simulink library "Valve_Lib"  (R2025a)
settings: Solver=ode45  StartTime=0.0  StopTime=10.0  RelTol=1e-3  EnableMultiTasking=on
libraries: fl_lib x13, Custom_lib x2, SimscapeFluids_lib x1
Description:
  | Copyright 2015-2025 The MathWorks, Inc.
settings Model: Creator=smiller  LastModifiedBy=smiller
settings SolverCC: AlgebraicLoopSolver=TrustRegion
settings DataIOCC: LimitDataPoints=on  SaveFormat=Array  ReturnWorkspaceOutputs=off
settings OptimizationCC: ReuseModelBlockBuffer=off  ExpressionDepthLimit=2147483647.0  LifeSpan=inf
settings DebuggingCC: UnderspecifiedInitializationDetection=Classic  MergeDetectMultiDrivingBlocksExec=none  SolverPrmCheckMsg=warning  UnconnectedInputMsg=warning  UnconnectedOutputMsg=warning  UnconnectedLineMsg=warning  AllowSymbolicDim=off  StateNameClashWarn=warning  PregeneratedLibrarySubsystemCodeDiagnostic=none  SFUnexpectedBacktrackingDiag=warning  SFNoUnconditionalDefaultTransitionDiag=warning  SFExecutionAtInitializationDiag=none  ArithmeticOperatorsInVariantConditions=warning
settings HardwareCC: ProdBitPerPointer=32.0  ProdBitPerSizeT=32.0  ProdBitPerPtrDiffT=32.0  ProdLargestAtomicFloat=None  ProdIntDivRoundTo=Undefined  ProdEndianess=Unspecified  ProdWordSize=32.0  ProdHWDeviceType=32-bit Generic
settings ModelReferenceCC: EnableRefExpFcnMdlSchedulingChecks=on  PropagateSignalLabelsOutOfModel=off
settings SFSimCC: SimUseLocalCustomCode=off  CustomCodeUndefinedFunction=UseInterfaceOnly
settings RTWCC: RTWUseLocalCustomCode=off  GPUComputeCapability=3.5  DLArmComputeVersion=19.05
settings CodeAppCC: StateflowObjectComments=on
settings GRTTargetCC: TargetLangStandard=C89/C90 (ANSI)
settings ConfigComp: CovMetricSettings=dw  CovSaveCumulativeToWorkspaceVar=on  CovSaveSingleToWorkspaceVar=on  CovExternalEMLEnable=off  CovSFcnEnable=off

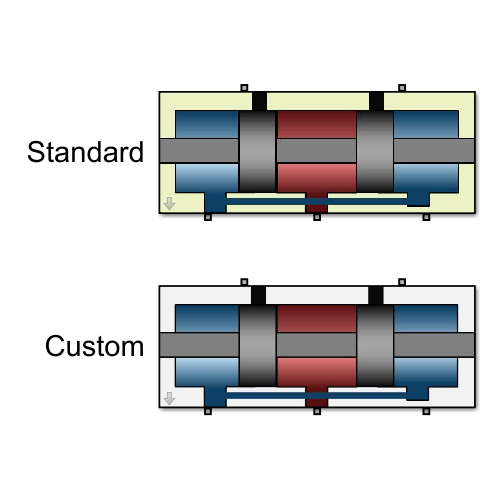
[thumbnail: Simulink's stored preview of the top-level diagram]
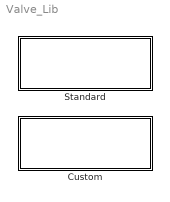
== system Valve_Lib ==
  Custom : Subsystem  VariantControl=Custom  mask(Single-Stage Servo Valve){K_V=0.5, x_max=0.5, A_max=9, x_lap=0.02, A_leak=0.25}
      mask prompts: K_V "Flow Coefficient:"; x_max "Spool travel limit (mm)"; A_max "Maximum orifice area (mm^2)"; x_lap "Spool travel with leakage (mm)"; A_leak "Leakage area at x=0 (mm^2)"
      mask help: Models a spool valve actuated directly by a torque motor using Simscape Foundation library components.
      mask Display: image('Four_Way_Valve_Custom_IMAGE.jpg')
  Standard : Subsystem  VariantControl=Standard  mask(Single-Stage Servo Valve){K_V=0.5, x_max=0.5, A_max=9, x_lap=0.02, A_leak=0.25}
      mask prompts: K_V "Flow Coefficient:"; x_max "Spool travel limit (mm)"; A_max "Maximum orifice area (mm^2)"; x_lap "Spool travel with leakage (mm)"; A_leak "Leakage area at x=0 (mm^2)"
      mask help: Models a spool valve actuated directly by a torque motor using Simscape add-on library components.
      mask Display: image(imread('Four_Way_Valve_Standard_IMAGE.jpg'))

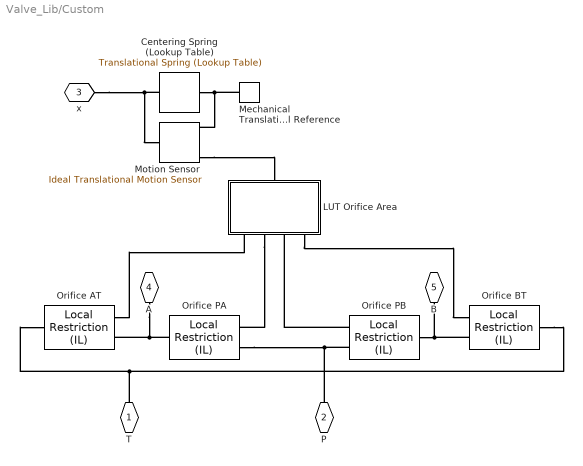
== system Valve_Lib/Custom ==
  Centering Spring (Lookup Table) : Custom_lib/Mechanical/Translational Spring (Lookup Table)  xd=[-1 -0.9 0,0.9 1]*x_max mm  kd=[100,10,10,10,100] N/m  f_specify=off  f_priority=High  f=0 N  f_nominal_specify=off  f_nominal_value=1  f_nominal_unit=N  x_specify=off  x_priority=High  x=0 m  x_nominal_specify=off  x_nominal_value=1  x_nominal_unit=m  v_specify=off  v_priority=High  v=0 m/s  v_nominal_specify=off  v_nominal_value=1  v_nominal_unit=m/s  k_specify=off  k_priority=High  k=0 N/m  k_nominal_specify=off  k_nominal_value=1  k_nominal_unit=N/m
      settings: InternalSimscapePortConfiguration="{\"Bottom\":[],\"Left\":[{\"id\":\"c\",\"label\":\"c\",\"type\":\"foundation.mechanical.translational.translational\"}],\"Right\":[{\"id\":\"r\",\"label\":\"r\",\"type\":\"foundation.mechanical.translational.translational\"}],\"Top\":[]}"
  LUT Orifice Area : Subsystem
  Mechanical Translational Reference : fl_lib/Mechanical/Translational Elements/Mechanical Translational Reference
  Motion Sensor : fl_lib/Mechanical/Mechanical Sensors/Ideal Translational Motion Sensor  reference=foundation.enum.MeasurementReference.difference  acceleration_port=false  velocity_port=true  position_port=true  offset=0 m
  Orifice AT : fl_lib/Isothermal Liquid/Elements/Local Restriction (IL)  restriction_type=foundation.enum.restriction_type.variable  restriction_area=1e-3 m^2  min_area=1e-12 m^2  max_area=1e10 m^2  area=inf m^2  Cd=K_V  Re_c=12  pressure_recovery=false
      settings: LibrarySourceBlock=fl_lib/Isothermal Liquid/Elements/Local Restriction (IL)  InternalSimscapePortConfiguration="{\"Bottom\":[],\"Left\":[{\"id\":\"A\",\"label\":\"A\",\"type\":\"foundation.isothermal_liquid.isothermal_liquid\"},{\"id\":\"AR\",\"label\":\"AR\",\"type\":\"input\"}],\"Right\":[{\"id\":\"B\",\"label\":\"B\",\"type\":\"foundation.isothermal_liquid.isothermal_liquid\"}],\"Top\":[]}"
  Orifice BT : fl_lib/Isothermal Liquid/Elements/Local Restriction (IL)  restriction_type=foundation.enum.restriction_type.variable  restriction_area=1e-3 m^2  min_area=1e-12 m^2  max_area=1e10 m^2  area=inf m^2  Cd=K_V  Re_c=12  pressure_recovery=false
      settings: LibrarySourceBlock=fl_lib/Isothermal Liquid/Elements/Local Restriction (IL)  InternalSimscapePortConfiguration="{\"Bottom\":[],\"Left\":[{\"id\":\"A\",\"label\":\"A\",\"type\":\"foundation.isothermal_liquid.isothermal_liquid\"},{\"id\":\"AR\",\"label\":\"AR\",\"type\":\"input\"}],\"Right\":[{\"id\":\"B\",\"label\":\"B\",\"type\":\"foundation.isothermal_liquid.isothermal_liquid\"}],\"Top\":[]}"
  Orifice PA : fl_lib/Isothermal Liquid/Elements/Local Restriction (IL)  restriction_type=foundation.enum.restriction_type.variable  restriction_area=1e-3 m^2  min_area=1e-12 m^2  max_area=1e10 m^2  area=inf m^2  Cd=K_V  Re_c=12  pressure_recovery=false
      settings: LibrarySourceBlock=fl_lib/Isothermal Liquid/Elements/Local Restriction (IL)  InternalSimscapePortConfiguration="{\"Bottom\":[],\"Left\":[{\"id\":\"A\",\"label\":\"A\",\"type\":\"foundation.isothermal_liquid.isothermal_liquid\"},{\"id\":\"AR\",\"label\":\"AR\",\"type\":\"input\"}],\"Right\":[{\"id\":\"B\",\"label\":\"B\",\"type\":\"foundation.isothermal_liquid.isothermal_liquid\"}],\"Top\":[]}"
  Orifice PB : fl_lib/Isothermal Liquid/Elements/Local Restriction (IL)  restriction_type=foundation.enum.restriction_type.variable  restriction_area=1e-3 m^2  min_area=1e-12 m^2  max_area=1e10 m^2  area=inf m^2  Cd=K_V  Re_c=12  pressure_recovery=false
      settings: LibrarySourceBlock=fl_lib/Isothermal Liquid/Elements/Local Restriction (IL)  InternalSimscapePortConfiguration="{\"Bottom\":[],\"Left\":[{\"id\":\"A\",\"label\":\"A\",\"type\":\"foundation.isothermal_liquid.isothermal_liquid\"},{\"id\":\"AR\",\"label\":\"AR\",\"type\":\"input\"}],\"Right\":[{\"id\":\"B\",\"label\":\"B\",\"type\":\"foundation.isothermal_liquid.isothermal_liquid\"}],\"Top\":[]}"
  T : PMIOPort  Tag=PMCPort  Side=Left
  P : PMIOPort  Tag=PMCPort  Port=2  Side=Left
  x : PMIOPort  Tag=PMCPort  Port=3  Side=Left
  A : PMIOPort  Tag=PMCPort  Port=4  Side=Right
  B : PMIOPort  Tag=PMCPort  Port=5  Side=Right
  connections:
  P/RConn1 -- Orifice PB/LConn1 -- Orifice PA/LConn1
  Mechanical Translational Reference/LConn1 -- Centering Spring (Lookup Table)/RConn1 -- Motion Sensor/RConn1
  x/RConn1 -- Centering Spring (Lookup Table)/LConn1 -- Motion Sensor/LConn1
  Motion Sensor/RConn3 -- LUT Orifice Area/LConn1
  Orifice AT/LConn2 -- LUT Orifice Area/RConn1
  Orifice PB/RConn1 -- Orifice BT/LConn1 -- B/RConn1
  Orifice PB/LConn2 -- LUT Orifice Area/RConn3
  T/RConn1 -- Orifice BT/RConn1 -- Orifice AT/RConn1
  A/RConn1 -- Orifice PA/RConn1 -- Orifice AT/LConn1
  LUT Orifice Area/RConn2 -- Orifice PA/LConn2
  LUT Orifice Area/RConn4 -- Orifice BT/LConn2

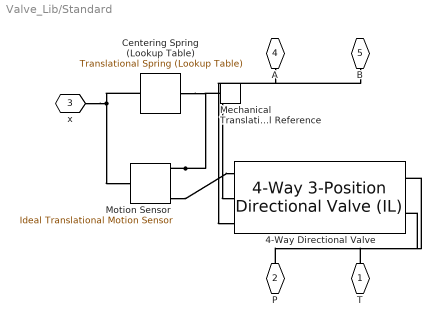
== system Valve_Lib/Standard ==
  4-Way Directional Valve : SimscapeFluids_lib/Isothermal Liquid/Valves & Orifices/Directional Control Valves/4-Way 3-Position Directional Valve (IL)  open_orifices_pos=fluids.isothermal_liquid.valves_orifices.directional_control_valves.enum.directional_valve_open_orifices_pos_neg.PA_BT  open_orifices_neu=fluids.isothermal_liquid.valves_orifices.directional_control_valves.enum.directional_valve_open_orifices_neutral.all_closed  open_orifices_neg=fluids.isothermal_liquid.valves_orifices.directional_control_valves.enum.directional_valve_open_orifices_pos_neg.PB_AT  neutral_assert_action=0  area_spec=fluids.isothermal_liquid.valves_orifices.directional_control_valves.enum.directional_valve_area_spec.identical  valve_spec=2  del_S_max=0.0049999 m  area_max=5e-5 m^2  del_S_TLU=[0 x_lap x_max]*1e-3 m  valve_area_TLU=[A_leak*0.1 A_leak A_max] mm^2  del_S_vol_flow_TLU=[0, .00125, .0025, .00375, .005] m  p_diff_TLU=[ -1e+7 -5e+6 -2e+6 2e+6 5e+6 1e+7 ] Pa  vol_flow_TLU=[ -1e-7 -7.0711e-8 -4.4721e-8 4.4721e-8 7.0711e-8 1e-7; -2.0352e-5 -1.4391e-5 -9.1017e-6 9.1017e-6 1.4391e-5 2.0352e-5; -0.0040736 -0.0028805 -0.0018218 0.0018218 0.0028805 0.0040736; -0.011438 -0.0080879 -0.0051152 0.0051152 0.0080879 0.011438; -0.034356 -0.024293 -0.015364 0.015364 0.024293 0.034356 ] m^3/s  p_diff_TLU_const=[-.1, .3, .5, .7] MPa  vol_flow_TLU_const=[-.0009, .0016, .002, .0024] m^3/s  area_const=1e-4 m^2  area_leak=1e-9 m^2  area=inf m^2  Cd=K_V  Re_c=12  smoothing_factor=0  pressure_recovery=false  S_max_PA=x_max mm  del_S_max_PA=0.0049999 m  area_max_PA=0.5e-4 m^2  del_S_TLU_PA=[-x_max -x_lap 0 x_lap x_max 2*x_max]*1e-3 m  valve_area_TLU_PA=[0 0 A_leak 2*A_leak A_max A_max] mm^2  del_S_vol_flow_TLU_PA=[0, .00125, .0025, .00375, .005] m  p_diff_TLU_PA=[-10000000.0, -5000000.0, -2000000.0, 2000000.0, 5000000.0, 10000000.0] Pa  vol_flow_TLU_PA=[-1.0e-7, -7.0711e-8, -4.4721e-8, 4.4721e-8, 7.0711e-8, 1.0e-7; -2.0352e-5, -1.4391e-5, -9.1017e-6, 9.1017e-6, 1.4391e-5, 2.0352e-5; -0.0040736, -0.0028805, -0.0018218, 0.0018218, 0.0028805, 0.0040736; -0.011438, -0.0080879, -0.0051152, 0.0051152, 0.0080879, 0.011438; -0.034356, -0.024293, -0.015364, 0.015364, 0.024293, 0.034356] m^3/s  area_const_PA=1e-4 m^2  p_diff_TLU_const_PA=[-.1, .3, .5, .7] MPa  vol_flow_TLU_const_PA=[-.0009, .0016, .002, .0024] m^3/s  S_max_PB=-x_max mm  del_S_max_PB=0.0049999 m  area_max_PB=0.5e-4 m^2  del_S_TLU_PB=[-x_max -x_lap 0 x_lap x_max 2*x_max]*1e-3 m  valve_area_TLU_PB=[0 0 A_leak 2*A_leak A_max A_max] mm^2  del_S_vol_flow_TLU_PB=[0, .00125, .0025, .00375, .005] m  p_diff_TLU_PB=[-10000000.0, -5000000.0, -2000000.0, 2000000.0, 5000000.0, 10000000.0] Pa  vol_flow_TLU_PB=[-1.0e-7, -7.0711e-8, -4.4721e-8, 4.4721e-8, 7.0711e-8, 1.0e-7; -2.0352e-5, -1.4391e-5, -9.1017e-6, 9.1017e-6, 1.4391e-5, 2.0352e-5; -0.0040736, -0.0028805, -0.0018218, 0.0018218, 0.0028805, 0.0040736; -0.011438, -0.0080879, -0.0051152, 0.0051152, 0.0080879, 0.011438; -0.034356, -0.024293, -0.015364, 0.015364, 0.024293, 0.034356] m^3/s  area_const_PB=1e-4 m^2  p_diff_TLU_const_PB=[-.1, .3, .5, .7] MPa  vol_flow_TLU_const_PB=[-.0009, .0016, .002, .0024] m^3/s  S_max_AB=7.5e-3 m  del_S_max_AB=0.005 m  area_max_AB=1e-4 m^2  del_S_TLU_AB=[0, .00125, .0025, .00375, .005] m  valve_area_TLU_AB=[1e-10, 1e-05, 4e-05, 6e-05, .0001] m^2  del_S_vol_flow_TLU_AB=[0, .00125, .0025, .00375, .005] m  p_diff_TLU_AB=[-.1, .3, .5, .7] MPa  vol_flow_TLU_AB=[-1e-08, 2.2e-08, 2.8e-08, 3.4e-08; -9e-06, .00015, .0002, .00024; -.00036, .00063, .00081, .00096; -.00054, .00094, .0012, .0014; -.00091, .0016, .002, .0024] m^3/s  area_const_AB=1e-4 m^2  p_diff_TLU_const_AB=[-.1, .3, .5, .7] MPa  vol_flow_TLU_const_AB=[-.0009, .0016, .002, .0024] m^3/s  S_max_AT=-x_max mm  del_S_max_AT=0.0049999 m  area_max_AT=0.5e-4 m^2  del_S_TLU_AT=[-x_max -x_lap 0 x_lap x_max 2*x_max]*1e-3 m  valve_area_TLU_AT=[0 0 A_leak 2*A_leak A_max A_max] mm^2  del_S_vol_flow_TLU_AT=[0, .00125, .0025, .00375, .005] m  p_diff_TLU_AT=[-10000000.0, -5000000.0, -2000000.0, 2000000.0, 5000000.0, 10000000.0] Pa  vol_flow_TLU_AT=[-1.0e-7, -7.0711e-8, -4.4721e-8, 4.4721e-8, 7.0711e-8, 1.0e-7; -2.0352e-5, -1.4391e-5, -9.1017e-6, 9.1017e-6, 1.4391e-5, 2.0352e-5; -0.0040736, -0.0028805, -0.0018218, 0.0018218, 0.0028805, 0.0040736; -0.011438, -0.0080879, -0.0051152, 0.0051152, 0.0080879, 0.011438; -0.034356, -0.024293, -0.015364, 0.015364, 0.024293, 0.034356] m^3/s  area_const_AT=1e-4 m^2  p_diff_TLU_const_AT=[-.1, .3, .5, .7] MPa  vol_flow_TLU_const_AT=[-.0009, .0016, .002, .0024] m^3/s  S_max_BT=x_max mm  del_S_max_BT=0.0049999 m  area_max_BT=0.5e-4 m^2  del_S_TLU_BT=[-x_max -x_lap 0 x_lap x_max 2*x_max]*1e-3 m  valve_area_TLU_BT=[0 0 A_leak 2*A_leak A_max A_max] mm^2  del_S_vol_flow_TLU_BT=[0, .00125, .0025, .00375, .005] m  p_diff_TLU_BT=[-10000000.0, -5000000.0, -2000000.0, 2000000.0, 5000000.0, 10000000.0] Pa  vol_flow_TLU_BT=[-1.0e-7, -7.0711e-8, -4.4721e-8, 4.4721e-8, 7.0711e-8, 1.0e-7; -2.0352e-5, -1.4391e-5, -9.1017e-6, 9.1017e-6, 1.4391e-5, 2.0352e-5; -0.0040736, -0.0028805, -0.0018218, 0.0018218, 0.0028805, 0.0040736; -0.011438, -0.0080879, -0.0051152, 0.0051152, 0.0080879, 0.011438; -0.034356, -0.024293, -0.015364, 0.015364, 0.024293, 0.034356] m^3/s  area_const_BT=1e-4 m^2  p_diff_TLU_const_BT=[-.1, .3, .5, .7] MPa  vol_flow_TLU_const_BT=[-.0009, .0016, .002, .0024] m^3/s  S_max_PT=0 m  del_S_max_PT=0.005 m  area_max_PT=1e-4 m^2  del_S_TLU_PT=[0, .00125, .0025, .00375, .005] m  valve_area_TLU_PT=[1e-10, 1e-05, 4e-05, 6e-05, .0001] m^2  del_S_vol_flow_TLU_PT=[0, .00125, .0025, .00375, .005] m  p_diff_TLU_PT=[-.1, .3, .5, .7] MPa  vol_flow_TLU_PT=[-1e-08, 2.2e-08, 2.8e-08, 3.4e-08; -9e-06, .00015, .0002, .00024; -.00036, .00063, .00081, .00096; -.00054, .00094, .0012, .0014; -.00091, .0016, .002, .0024] m^3/s
      settings: LibrarySourceBlock=SimscapeFluids_lib/Isothermal Liquid/Valves & Orifices/Directional Control Valves/4-Way 3-Position Directional Valve (IL)  InternalSimscapePortConfiguration="{\"Bottom\":[{\"id\":\"P\",\"label\":\"P\",\"type\":\"foundation.isothermal_liquid.isothermal_liquid\"},{\"id\":\"T\",\"label\":\"T\",\"type\":\"foundation.isothermal_liquid.isothermal_liquid\"}],\"Left\":[{\"id\":\"S\",\"label\":\"S\",\"type\":\"input\"}],\"Right\":[],\"Top\":[{\"id\":\"A\",\"label\":\"A\",\"type\":\"foundation.isothermal_liquid.isothermal_liquid\"},{\"id\":\"B\",\"label\":\"B\",\"type\":\"foundation.isothermal_liquid.isothermal_liquid\"}]}"
  Centering Spring (Lookup Table) : Custom_lib/Mechanical/Translational Spring (Lookup Table)  xd=[-1 -0.9 0,0.9 1]*x_max mm  kd=[100,10,10,10,100] N/m  f_specify=off  f_priority=High  f=0 N  f_nominal_specify=off  f_nominal_value=1  f_nominal_unit=N  x_specify=off  x_priority=High  x=0 m  x_nominal_specify=off  x_nominal_value=1  x_nominal_unit=m  v_specify=off  v_priority=High  v=0 m/s  v_nominal_specify=off  v_nominal_value=1  v_nominal_unit=m/s  k_specify=off  k_priority=High  k=0 N/m  k_nominal_specify=off  k_nominal_value=1  k_nominal_unit=N/m
      settings: InternalSimscapePortConfiguration="{\"Bottom\":[],\"Left\":[{\"id\":\"c\",\"label\":\"c\",\"type\":\"foundation.mechanical.translational.translational\"}],\"Right\":[{\"id\":\"r\",\"label\":\"r\",\"type\":\"foundation.mechanical.translational.translational\"}],\"Top\":[]}"
  Mechanical Translational Reference : fl_lib/Mechanical/Translational Elements/Mechanical Translational Reference
  Motion Sensor : fl_lib/Mechanical/Mechanical Sensors/Ideal Translational Motion Sensor  reference=foundation.enum.MeasurementReference.difference  acceleration_port=false  velocity_port=true  position_port=true  offset=0 m
  T : PMIOPort  Tag=PMCPort  Side=Left
  P : PMIOPort  Tag=PMCPort  Port=2  Side=Left
  x : PMIOPort  Tag=PMCPort  Port=3  Side=Left
  A : PMIOPort  Tag=PMCPort  Port=4  Side=Right
  B : PMIOPort  Tag=PMCPort  Port=5  Side=Right
  connections:
  Motion Sensor/RConn1 -- Centering Spring (Lookup Table)/RConn1 -- Mechanical Translational Reference/LConn1
  x/RConn1 -- Centering Spring (Lookup Table)/LConn1 -- Motion Sensor/LConn1
  Motion Sensor/RConn3 -- 4-Way Directional Valve/LConn1
  A/RConn1 -- 4-Way Directional Valve/LConn2
  B/RConn1 -- 4-Way Directional Valve/LConn3
  T/RConn1 -- 4-Way Directional Valve/RConn2
  P/RConn1 -- 4-Way Directional Valve/RConn1

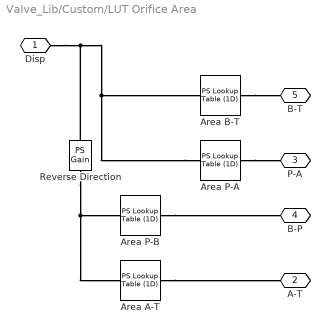
== system Valve_Lib/Custom/LUT Orifice Area ==
  Area A-T : fl_lib/Physical Signals/Lookup Tables/PS Lookup Table (1D)  x=[-x_max -x_lap 0 x_lap x_max 2*x_max]*1e-3 m  f=[0 0 A_leak 2*A_leak A_max A_max]*1e-6 m^2  interp_method=simscape.enum.interpolation.linear  extrap_method=simscape.enum.extrapolation.linear
  Area B-T : fl_lib/Physical Signals/Lookup Tables/PS Lookup Table (1D)  x=[-x_max -x_lap 0 x_lap x_max 2*x_max]*1e-3 m  f=[0 0 A_leak 2*A_leak A_max A_max]*1e-6 m^2  interp_method=simscape.enum.interpolation.linear  extrap_method=simscape.enum.extrapolation.linear
  Area P-A : fl_lib/Physical Signals/Lookup Tables/PS Lookup Table (1D)  x=[-x_max -x_lap 0 x_lap x_max 2*x_max]*1e-3 m  f=[0 0 A_leak 2*A_leak A_max A_max]*1e-6 m^2  interp_method=simscape.enum.interpolation.linear  extrap_method=simscape.enum.extrapolation.linear
  Area P-B : fl_lib/Physical Signals/Lookup Tables/PS Lookup Table (1D)  x=[-x_max -x_lap 0 x_lap x_max 2*x_max]*1e-3 m  f=[0 0 A_leak 2*A_leak A_max A_max]*1e-6 m^2  interp_method=simscape.enum.interpolation.linear  extrap_method=simscape.enum.extrapolation.linear
  Reverse Direction : fl_lib/Physical Signals/Functions/PS Gain  gain=-1
  Disp : PMIOPort  Side=Left
  A-T : PMIOPort  Port=2  Side=Right
  P-A : PMIOPort  Port=3  Side=Right
  B-P : PMIOPort  Port=4  Side=Right
  B-T : PMIOPort  Port=5  Side=Right
  connections:
  Area P-A/RConn1 -- P-A/RConn1
  Area P-A/LConn1 -- Area B-T/LConn1 -- Reverse Direction/LConn1 -- Disp/RConn1
  Area B-T/RConn1 -- B-T/RConn1
  Reverse Direction/RConn1 -- Area P-B/LConn1 -- Area A-T/LConn1
  Area P-B/RConn1 -- B-P/RConn1
  Area A-T/RConn1 -- A-T/RConn1
